simulink model "function_temp_sensor"  (R2023b)
settings: Solver=FixedStepDiscrete  StartTime=0.0  StopTime=10.0  FixedStep=0.01  RelTol=1e-3
settings Model: Creator=levadny  LastModifiedBy=frost
settings DataIOCC: SaveOutput=off  SaveTime=off
settings OptimizationCC: DefaultParameterBehavior=Inlined  EnhancedBackFolding=on  PassReuseOutputArgsAs=Individual arguments  ZeroExternalMemoryAtStartup=off  ZeroInternalMemoryAtStartup=off  OptimizeBlockOrder=speed  DifferentSizesBufferReuse=on  OptimizationCustomize=off  EfficientTunableParamExpr=on
settings DebuggingCC: ParameterTunabilityLossMsg=error
settings SFSimCC: MATLABDynamicMemAlloc=off
settings RTWCC: Description=Embedded Coder  SystemTargetFile=ert.tlc  TemplateMakefile=ert_default_tmf  GenerateReport=on
settings CodeAppCC: ForceParamTrailComments=on  IgnoreCustomStorageClasses=off  OperatorAnnotations=on  SimulinkDataObjDesc=on  SFDataObjDesc=on  InsertBlockDesc=on
settings ERTTargetCC: TargetLangStandard=C99 (ISO)  GenerateSampleERTMain=on  InlinedParameterPlacement=NonHierarchical  ERTCustomFileTemplate=example_file_process.tlc

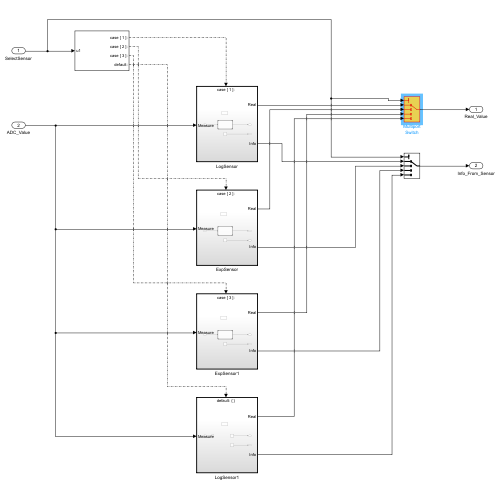
[thumbnail: Simulink's stored preview of the top-level diagram]
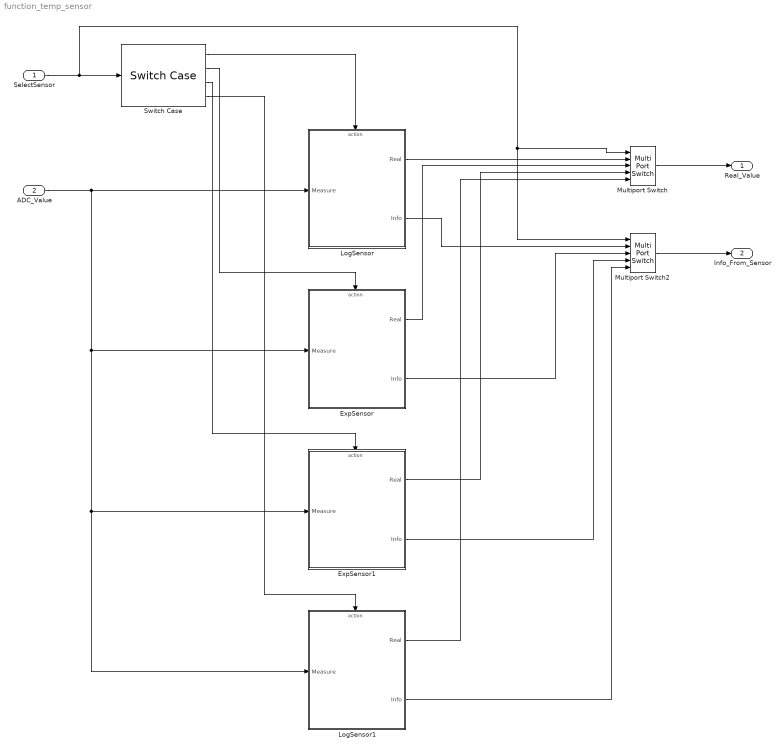
== system function_temp_sensor ==
  SelectSensor : Inport  OutDataTypeStr=int8
  ADC_Value : Inport  Port=2  OutDataTypeStr=double
  ExpSensor : Subsystem  TreatAsAtomicUnit=on
  ExpSensor1 : Subsystem  TreatAsAtomicUnit=on
  LogSensor : Subsystem  TreatAsAtomicUnit=on
  LogSensor1 : Subsystem  TreatAsAtomicUnit=on
  Multiport Switch : MultiPortSwitch  Inputs=4  DiagnosticForDefault=None  SaturateOnIntegerOverflow=off  InputSameDT=off
  Multiport Switch2 : MultiPortSwitch  Inputs=4  SaturateOnIntegerOverflow=off  InputSameDT=off
  Switch Case : SwitchCase  CaseConditions={1, 2, 3}
  Real_Value : Outport  OutDataTypeStr=double
  Info_From_Sensor : Outport  Port=2  OutDataTypeStr=int8
  wires:
  ADC_Value/1 -> LogSensor1/1(Measure), ExpSensor1/1(Measure), ExpSensor/1(Measure), LogSensor/1(Measure)
  SelectSensor/1 -> Multiport Switch2/1, Multiport Switch/1, Switch Case/1
  Multiport Switch/1 -> Real_Value/1
  Switch Case/4 -> LogSensor1/Action
  Multiport Switch2/1 -> Info_From_Sensor/1
  Switch Case/1 -> LogSensor/Action
  Switch Case/2 -> ExpSensor/Action
  LogSensor/1(Real) -> Multiport Switch/2
  ExpSensor/1(Real) -> Multiport Switch/3
  ExpSensor1/1(Real) -> Multiport Switch/4
  ExpSensor1/2(Info) -> Multiport Switch2/4
  ExpSensor/2(Info) -> Multiport Switch2/3
  LogSensor/2(Info) -> Multiport Switch2/2
  Switch Case/3 -> ExpSensor1/Action
  LogSensor1/1(Real) -> Multiport Switch/5
  LogSensor1/2(Info) -> Multiport Switch2/5

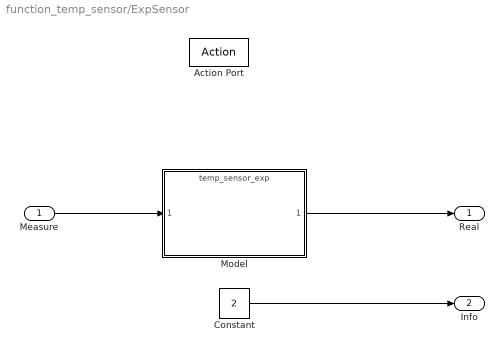
== system function_temp_sensor/ExpSensor ==
  Measure : Inport  OutDataTypeStr=double
  Action Port : ActionPort  ActionPortLabel=case [ 2 ]:
  Constant : Constant  Value=2  OutDataTypeStr=int8
  Model : ModelReference  ModelNameDialog=temp_sensor_exp.slx  SimulationMode=Normal  ModelReferenceVersion=1.10
  Real : Outport  OutDataTypeStr=double
  Info : Outport  Port=2  OutDataTypeStr=int8
  wires:
  Constant/1 -> Info/1
  Measure/1 -> Model/1
  Model/1 -> Real/1

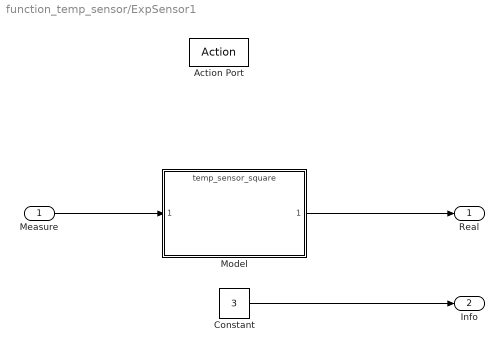
== system function_temp_sensor/ExpSensor1 ==
  Measure : Inport  OutDataTypeStr=double
  Action Port : ActionPort  ActionPortLabel=case [ 3 ]:
  Constant : Constant  Value=3  OutDataTypeStr=int8
  Model : ModelReference  ModelNameDialog=temp_sensor_square.slx  SimulationMode=Normal  ModelReferenceVersion=1.9
  Real : Outport  OutDataTypeStr=double
  Info : Outport  Port=2  OutDataTypeStr=int8
  wires:
  Constant/1 -> Info/1
  Measure/1 -> Model/1
  Model/1 -> Real/1

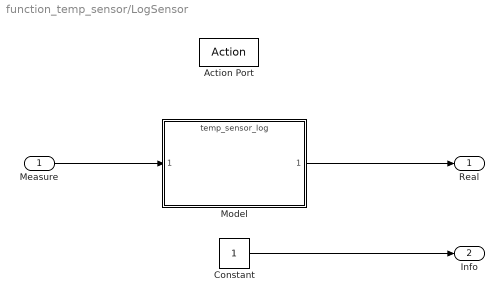
== system function_temp_sensor/LogSensor ==
  Measure : Inport  OutDataTypeStr=double
  Action Port : ActionPort  ActionPortLabel=case [ 1 ]:
  Constant : Constant  OutDataTypeStr=int8
  Model : ModelReference  ModelNameDialog=temp_sensor_log.slx  SimulationMode=Normal  ModelReferenceVersion=1.7
  Real : Outport  OutDataTypeStr=double
  Info : Outport  Port=2  OutDataTypeStr=int8
  wires:
  Model/1 -> Real/1
  Measure/1 -> Model/1
  Constant/1 -> Info/1

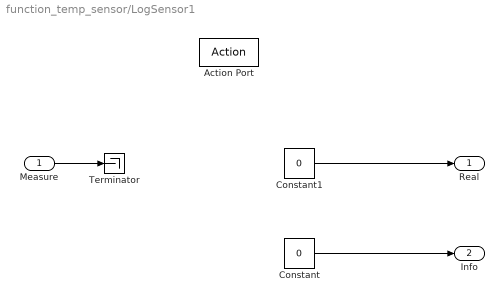
== system function_temp_sensor/LogSensor1 ==
  Measure : Inport  OutDataTypeStr=double
  Action Port : ActionPort  ActionPortLabel=default:
  Constant : Constant  Value=0  OutDataTypeStr=int8
  Constant1 : Constant  Value=0  OutDataTypeStr=double
  Terminator : Terminator
  Real : Outport  OutDataTypeStr=double
  Info : Outport  Port=2  OutDataTypeStr=int8
  wires:
  Constant1/1 -> Real/1
  Measure/1 -> Terminator/1
  Constant/1 -> Info/1
